simulink model "HT_ctrl_MPC_23"  (R2023a)
settings: Solver=VariableStepAuto  StartTime=0.0  StopTime=50  FixedStep=1  RelTol=1e-3
undefined symbols (not defined in the file): D1, Delta, robust_actuator_gain_scale, robust_actuator_rate_limit, robust_actuator_time_constant, robust_load_switch_time, robust_measurement_delay_s, robust_noise_seed, robust_noise_std
libraries: spsThreePhaseParallelRLCLoadLib x3, spsExcitationSystemModel x2, spsThreePhaseSourceLib x1, simulink x1, spsSynchronousMachinepuStandardLib x1, spsThreePhaseBreakerLib x1, spsThreePhaseTransformerTwoWindingsLib x1, spsVoltageMeasurementLib x1, spsGroundLib x1, spspowerguiLib x1
Description:
  | Phase-2.3 filtered, disturbance-estimating MPC with soft output constraints and anti-windup; generated from phase-2 harness.
settings Model: Creator=zzzaa  LastModifiedBy=User
settings OptimizationCC: ReuseModelBlockBuffer=off

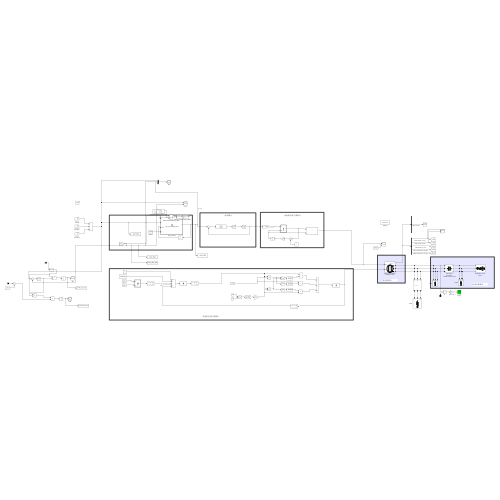
[thumbnail: Simulink's stored preview of the top-level diagram]
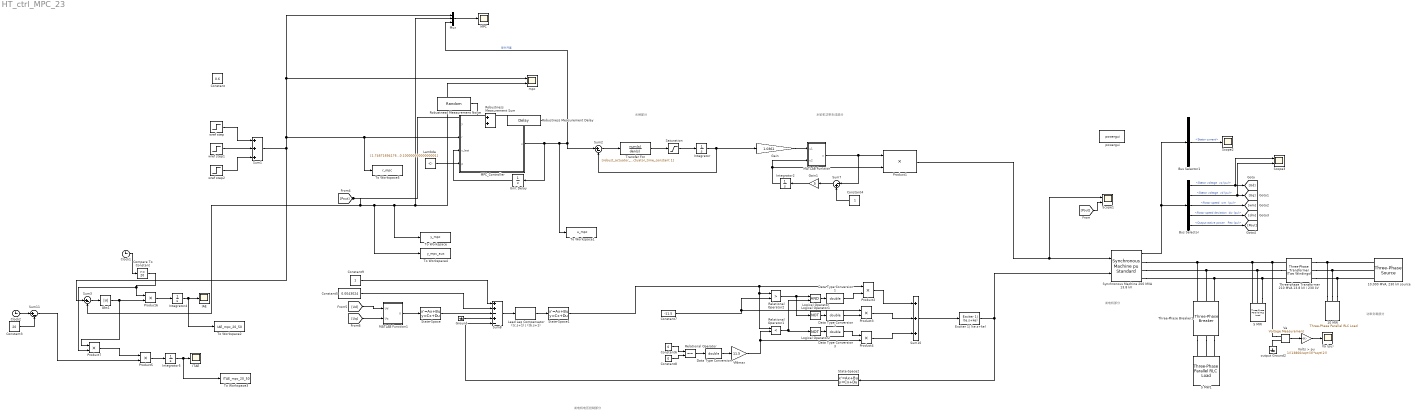
== system HT_ctrl_MPC_23 ==
  note: 水轮机功率生成部分
  note: 水闸部分
  note: 发电机电压控制部分
  note: 发电机部分
  note: 功率负载部分
  10 MW : spsThreePhaseParallelRLCLoadLib/Three-Phase Parallel RLC Load  LConnTagsString=A|B|C  Configuration=Y (grounded)  NominalVoltage=230e3  Vabc=[1e3 1e3 1e3]  Vabcp=[1e3 1e3 1e3]  NominalFrequency=60  UnbalancedPower=off  ActivePower=10000000  InductivePower=0  CapacitivePower=0  Pabc=[10e3 9e3 11e3]  QLabc=[100 90 110]  QCabc=[100 90 110]  Pabcp=[10e3 9e3 11e3]  QLabcp=[100 90 110]  QCabcp=[100 90 110]  Measurements=None  LoadType=constant Z
  "10,000 MVA, 230 kV source" : spsThreePhaseSourceLib/Three-Phase Source  InternalConnection=Yg  VoltagePhases=off  Voltage=(230000)*1.00006  PhaseAngle=-0.77547  Voltage_phases=[25e3 25e3 25e3]/sqrt(3)  PhaseAngles_phases=[0 -120 +120]  Frequency=60  NonIdealSource=on  SpecifyImpedance=on  Resistance=0.529  Inductance=0.0140  ShortCircuitLevel=10000e6  BaseVoltage=230e3  XRratio=10  BusType=swing  Pref=0  Qref=0  Prefabc=[10e3, 10e3, 10e3]  Qrefabc=[0, 0, 0]  Qmin=-Inf  Qmax=Inf
  5 MW : spsThreePhaseParallelRLCLoadLib/Three-Phase Parallel RLC Load  LConnTagsString=A|B|C  Configuration=Y (grounded)  NominalVoltage=13.8e3  Vabc=[1e3 1e3 1e3]  Vabcp=[1e3 1e3 1e3]  NominalFrequency=60  UnbalancedPower=off  ActivePower=5000000  InductivePower=0  CapacitivePower=0  Pabc=[10e3 9e3 11e3]  QLabc=[100 90 110]  QCabc=[100 90 110]  Pabcp=[10e3 9e3 11e3]  QLabcp=[100 90 110]  QCabcp=[100 90 110]  Measurements=None  LoadType=constant Z
  5 MW1 : spsThreePhaseParallelRLCLoadLib/Three-Phase Parallel RLC Load  LConnTagsString=A|B|C  Configuration=Y (grounded)  NominalVoltage=13.8e3  Vabc=[1e3 1e3 1e3]  Vabcp=[1e3 1e3 1e3]  NominalFrequency=60  UnbalancedPower=off  ActivePower=robust_load_power_w  InductivePower=0  CapacitivePower=0  Pabc=[10e3 9e3 11e3]  QLabc=[100 90 110]  QCabc=[100 90 110]  Pabcp=[10e3 9e3 11e3]  QLabcp=[100 90 110]  QCabcp=[100 90 110]  Measurements=None  LoadType=constant Z
  Abs1 : Abs  ZeroCross=off  SaturateOnIntegerOverflow=off
  Bus Selector : BusSelector  OutputSignals="dq0 components.Stator voltage  vq (pu),dq0 components.Stator voltage  vd (pu),Mechanical.Rotor speed  wm  (pu),Mechanical.Rotor speed deviation  dw (pu),Output active power   Peo (pu)"
  Bus Selector1 : BusSelector  OutputSignals=Stator current
  Clock1 : Clock
  Clock2 : Clock
  Compare To Constant : simulink/Logic and Bit Operations/Compare To Constant  relop=>=  const=20  OutDataTypeStr=boolean
  Constant : Constant  Value=0.6
  Constant3 : Constant  Value=20
  Constant4 : Constant
  Constant5 : Constant  Value=0.0043024
  Constant6 : Constant  Value=0
  Constant7 : Constant  Value=-11.5
  Constant8 : Constant  Value=0
  Constant9 : Constant
  Data Type Conversion{,1..3} (4 alike) : DataTypeConversion  OutDataTypeStr=double  SaturateOnIntegerOverflow=off  RndMeth=Floor
  Exciter 1| (te.s+ke) : spsExcitationSystemModel/Continuous/Exciter 1| (te.s+ke)  N=1  D=[0 1]  Y0=1.2907  U0=1.2907
  Gain : Gain  Gain=1.0361
  Gain1 : Gain  Gain=5
  Ground : Ground
  IAE : Scope
  ITAE : Scope
  Integrator : Integrator  InitialCondition=0.72544  LimitOutput=on  UpperSaturationLimit=0.97518  LowerSaturationLimit=0.01
  Integrator2 : Integrator  InitialCondition=0.75161
  Integrator4 : Integrator
  Integrator5 : Integrator
  Lambda : Constant  Value=[1.7467169417629138 -0.75577185457135487 0.064765752859370848 -0.055077765078686149 -0.00021442550980328465 1 40 0.014999999999999999 -1.1499999999999999 1.1499999999999999 0.029999999999999999 0.029999999999999999 0.02 0.10000000000000001 0.050000000000000003 0.02 0.34999999999999998 1 20 0.10000000000000001]
  Lead Lag Compensator (tc.s+1) | (tb.s+1) : spsExcitationSystemModel/Continuous/Lead Lag Compensator (tc.s+1) | (tb.s+1)  N=[0 1]  D=[0 1]  Y0=0.0043024  U0=0.0043024
  Logical Operator : Logic
  Logical Operator1 : Logic  Operator=NOT  Inputs=1
  Logical Operator2 : Logic  Operator=NOT  Inputs=1
  MATLAB Function : MATLAB Function  TreatAsAtomicUnit=on
  MATLAB Function1 : MATLAB Function  TreatAsAtomicUnit=on
  MPC : Scope
  MPC_Controller : MATLAB Function  TreatAsAtomicUnit=on  SystemSampleTime=0.01
  Mux : Mux  Inputs=3
  Product{1,5..7} (4 alike) : Product
  Product2 : Product  InputSameDT=on  SaturateOnIntegerOverflow=on  OutDataTypeStr=Inherit: Same as first input
  Product3 : Product  InputSameDT=on  SaturateOnIntegerOverflow=on  OutDataTypeStr=Inherit: Same as first input
  Product4 : Product  InputSameDT=on  SaturateOnIntegerOverflow=on  OutDataTypeStr=Inherit: Same as first input
  Relational Operator : RelationalOperator  Operator===
  Relational Operator1 : RelationalOperator  Operator=<
  Relational Operator2 : RelationalOperator  Operator=>
  Robustness Measurement Delay : TransportDelay  DelayTime=robust_measurement_delay_s  InitialOutput=0.5
  Robustness Measurement Noise : RandomNumber  Variance=robust_noise_std^2  Seed=robust_noise_seed  SampleTime=0.01
  Robustness Measurement Sum : Sum
  Saturation : Saturate  UpperLimit=robust_actuator_rate_limit  LowerLimit=-robust_actuator_rate_limit
  Scope1 : Scope  NumInputPorts=2
  Scope2 : Scope
  Scope3 : Scope  NumInputPorts=2
  State-Space : StateSpace  A=-50  C=50  D=0  InitialCondition=0.02
  State-Space1 : StateSpace  A=-1000  C=300000  D=0  InitialCondition=4.3024e-6
  State-Space2 : StateSpace  A=-10  C=-0.1  D=0.01  InitialCondition=0.1297
  Sum1 : Sum  Inputs=+++  InputSameDT=on  SaturateOnIntegerOverflow=on  OutDataTypeStr=Inherit: Same as first input
  Sum10 : Sum  Inputs=+++  InputSameDT=on  SaturateOnIntegerOverflow=on  OutDataTypeStr=Inherit: Same as first input
  Sum11 : Sum  Inputs=|+-
  Sum2 : Sum  Inputs=|+-
  Sum3 : Sum  Inputs=|+-
  Sum7 : Sum  Inputs=|-+
  Sum8 : Sum  Inputs=++-+-  InputSameDT=on  SaturateOnIntegerOverflow=on  OutDataTypeStr=Inherit: Same as first input
  Synchronous Machine 200 MVA 13.8 kV : spsSynchronousMachinepuStandardLib/Synchronous Machine pu Standard  PresetModel=No  MechanicalLoad=Mechanical power Pm  ShowDetailedParameters=on  RotorType=Salient-pole  Units=per unit standard parameters  MeasurementBus=off  NominalParameters="[ 200E6  13800   60 ]"  Reactances1=[ 31 32 33 34 35 36 37 ]  Reactances2=[ 1.305, 0.296, 0.252, 0.474, 0.243, 0.18 ]  dAxisTimeConstants=Short-circuit  qAxisTimeConstants=Open-circuit  TimeConstants1=[]  TimeConstants2=[]  TimeConstants3=[]  TimeConstants4=[]  TimeConstants5=[ 1.01, 0.053, 0.1 ]  TimeConstants6=[]  TimeConstants7=[]  TimeConstants8=[]  StatorResistance=2.8544e-3  Mechanical=[ 3.2 0 2]  PolePairs=2  InitialConditions=[0 -94.2826 0.750185 0.750185 0.750185 -24.943 -144.943 95.057 1.29071]  SetSaturation=off  Saturation=[0.6404,0.7127,0.8441,0.9214,0.9956,1.082,1.19,1.316,1.457;0.7,0.7698,0.8872,0.9466,0.9969,1.046,1.1,1.151,1.201]  LoadFlowParameters=[1 150000000 0 0]  TsPowergui=0  TsBlock=-1  IterativeModel=Trapezoidal non iterative  IterativeDiscreteModel=Trapezoidal non iterative  BusType=PV  Pref=150000000  Qref=0  Qmin=-Inf  Qmax=Inf  PLF=0  QLF=0
  Three-Phase Breaker1 : spsThreePhaseBreakerLib/Three-Phase Breaker  InitialState=open  SwitchA=on  SwitchB=on  SwitchC=on  SwitchTimes=[robust_load_switch_time]  External=off  BreakerResistance=0.01  SnubberResistance=1e6  SnubberCapacitance=inf  Measurements=None
  Three-phase Transformer 210 MVA 13.8 kV / 230 kV : spsThreePhaseTransformerTwoWindingsLib/Three-Phase Transformer (Two Windings)  Winding1Connection=Delta (D1)  Winding2Connection=Yg  CoreType=Three single-phase transformers  SetSaturation=off  Hysteresis=off  DataFile='hysteresis'  SetInitialFlux=off  Measurements=None  UNITS=pu  NominalPower=[ 210e6 60 ]  Winding1="[ 13.8e3 0.0027  0.08]"  Winding2=[ 230e3 0.0027 0.08]  Rm=500  Lm=500  L0=0.5  Saturation="[ 0,0  ;  0.005,1.2  ;  1.0,1.4 ]"  InitialFluxes=[ 0.8 , -0.8 , 0.7 ]  BreakLoop=off  DiscreteSolver=Trapezoidal iterative  DataType=off  TransfoNumber=0
  To Workspace : ToWorkspace  VariableName=y_mpc  SampleTime=-1
  To Workspace1 : ToWorkspace  VariableName=u_mpc  SampleTime=-1
  To Workspace2 : ToWorkspace  VariableName=IAE_mpc_20_50  SampleTime=-1
  To Workspace3 : ToWorkspace  VariableName=ITAE_mpc_20_50  SampleTime=-1
  To Workspace4 : ToWorkspace  VariableName=y_mpc_aux  SampleTime=-1
  To Workspace5 : ToWorkspace  VariableName=r_mpc  SampleTime=-1
  Transfer Fcn : TransferFcn  Numerator=[robust_actuator_gain_scale*10/3]  Denominator=[robust_actuator_time_constant 1]
  Unit Delay : UnitDelay  SampleTime=0.01  HasFrameUpgradeWarning=on
  Va : spsVoltageMeasurementLib/Voltage Measurement  Tag=PoWeRsYsTeMmEaSuReMeNt  PhasorSimulation=off  OutputType=Magnitude  PSBequivalent=0
  Va (pu) : Scope
  Vfdmax : Gain  Gain=11.5  SaturateOnIntegerOverflow=on  OutDataTypeStr=Inherit: Same as input  ParamDataTypeStr=Inherit: Same as input
  Volts > pu : Gain  Gain=1/(13800/sqrt(3)*sqrt(2))  SaturateOnIntegerOverflow=on  OutDataTypeStr=Inherit: Same as input  ParamDataTypeStr=Inherit: Same as input
  mpc : Scope  NumInputPorts=2
  output Ground2 : spsGroundLib/Ground  LConnTagsString=a
  powergui : spspowerguiLib/powergui  Priority=2  SimulationMode=Continuous  SampleTime=0  frequency=60  Iterations=50  frequencyindice=60  Pbase=100e6  ErrMax=0.0001  UnitsV=kV  UnitsW=MW  buscounter=0  FunctionMessages=off  echomessages=off  EnableUseOfTLC=off  CurrentSourceSwitches=off  DisableSnubberDevices=off  DisableRonSwitches=off  DisableVfSwitches=off  DisplayEquations=off  AutomaticDiscreteSolvers=off  SolverType=Tustin  Interpol=off  ExternalGateDelay=off  methode=off  Ts=0  x0status=blocks  SPID=on  SwTol=0  HookPort=off  NonlinearTolerance=0  nMaxIteration=15  ContinueOnMaxIteration=off  RestoreLinks=warning  ResistiveCurrentMeasurement=off  Frange=logspace(0,3,50)  Ylog=off  Xlog=off  ShowGrid=off  save=off  variable=ZData  structure=0  ZoomFFT=on  StartTime=0.0  cycles=2  DisplayStyle=off  fundamental=60  FreqAxis=off  MaxFrequency=1000  frequencyindicesteady=1  RmsSteady=1  display=off
  wref step : Step  Time=0  After=0.5  SampleTime=0
  wref step1 : Step  Time=20  After=0.25  SampleTime=0
  wref step2 : Step  Time=35  After=0.15  SampleTime=0
  wires:
  Va/1 -> Volts > pu/1
  Volts > pu/1 -> Va (pu)/1
  Synchronous Machine 200 MVA 13.8 kV/1 -> Bus Selector1/1, Bus Selector/1
  Bus Selector/1 -> Scope3/1, [Ud]  "<Stator voltage  vq (pu)>"
  Bus Selector/2 -> Scope3/2, [Uq]  "<Stator voltage  vd (pu)>"
  Bus Selector/3 -> [wm]  "<Rotor speed  wm  (pu)>"
  Bus Selector/4 -> [dm]  "<Rotor speed deviation  dw (pu)>"
  Bus Selector/5 -> [Pout]  "<Output active power   Peo (pu)>"
  MPC_Controller/1(u) -> To Workspace1/1, Sum2/1, Mux/3, Unit Delay/1  "导叶开度"
  Transfer Fcn/1 -> Saturation/1
  Saturation/1 -> Integrator/1
  Sum2/1 -> Transfer Fcn/1
  Gain/1 -> MATLAB Function/1(u1)
  MATLAB Function/1(y) -> Product1/1, Sum7/1
  Constant4/1 -> Sum7/2
  Sum7/1 -> Gain1/1
  Gain1/1 -> Integrator2/1
  Integrator2/1 -> MATLAB Function/2(u2), Product1/2
  State-Space2/1 -> Sum8/5
  Exciter 1| (te.s+ke)/1 -> Synchronous Machine 200 MVA 13.8 kV/2, State-Space2/1
  MATLAB Function1/1(U) -> State-Space/1
  Lead Lag Compensator (tc.s+1) | (tb.s+1)/1 -> State-Space1/1
  [Ud] -> MATLAB Function1/1(Ud)
  Constant5/1 -> Sum8/2
  Constant9/1 -> Sum8/1
  Sum10/1 -> Exciter 1| (te.s+ke)/1
  [Uq] -> MATLAB Function1/2(Uq)
  Sum8/1 -> Lead Lag Compensator (tc.s+1) | (tb.s+1)/1
  Ground/1 -> Sum8/4
  Logical Operator2/1 -> Data Type Conversion3/1
  State-Space/1 -> Sum8/3
  Constant6/1 -> Relational Operator/1
  Product2/1 -> Sum10/1
  Constant8/1 -> Relational Operator/2
  Product4/1 -> Sum10/3
  Relational Operator1/1 -> Logical Operator2/1, Logical Operator/2
  Product3/1 -> Sum10/2
  Constant7/1 -> Product3/1, Relational Operator2/2
  Relational Operator2/1 -> Logical Operator1/1, Logical Operator/1
  Logical Operator/1 -> Data Type Conversion1/1
  Vfdmax/1 -> Product4/2, Relational Operator1/2
  State-Space1/1 -> Product2/1, Relational Operator1/1, Relational Operator2/1
  Data Type Conversion/1 -> Vfdmax/1
  Data Type Conversion1/1 -> Product2/2
  Data Type Conversion2/1 -> Product3/2
  Logical Operator1/1 -> Data Type Conversion2/1
  Data Type Conversion3/1 -> Product4/1
  Relational Operator/1 -> Data Type Conversion/1
  Product1/1 -> Scope1/1, Synchronous Machine 200 MVA 13.8 kV/1
  Bus Selector1/1 -> Scope2/1  "<Stator current>"
  [Pout] -> Scope1/2
  wref step/1 -> Sum1/1
  wref step1/1 -> Sum1/2
  wref step2/1 -> Sum1/3
  Mux/1 -> MPC/1
  Integrator/1 -> Sum2/2, Gain/1
  Unit Delay/1 -> MPC_Controller/3(u_last)
  Clock1/1 -> Compare To Constant/1
  Compare To Constant/1 -> Product7/2, Product6/1
  Clock2/1 -> Sum11/1
  Product7/1 -> Product5/1
  Sum11/1 -> Product5/2
  Product6/1 -> Integrator4/1
  Constant3/1 -> Sum11/2
  Sum3/1 -> Abs1/1
  Integrator4/1 -> To Workspace2/1, IAE/1
  Sum1/1 -> Sum3/1, mpc/1, Mux/1, MPC_Controller/2(r), To Workspace5/1
  Product5/1 -> Integrator5/1
  Integrator5/1 -> To Workspace3/1, ITAE/1
  [Pout] -> Sum3/2, To Workspace4/1, To Workspace/1, Mux/2, mpc/2, Robustness Measurement Sum/1
  Abs1/1 -> Product7/1, Product6/2
  Lambda/1 -> MPC_Controller/4(p)
  Robustness Measurement Noise/1 -> Robustness Measurement Sum/2
  Robustness Measurement Sum/1 -> Robustness Measurement Delay/1
  Robustness Measurement Delay/1 -> MPC_Controller/1(y)
  connections:
  10 MW/LConn2 -- Three-phase Transformer 210 MVA 13.8 kV / 230 kV/RConn2 -- "10,000 MVA, 230 kV source"/RConn2
  Va/LConn1 -- Three-Phase Breaker1/LConn1 -- Synchronous Machine 200 MVA 13.8 kV/RConn1 -- 5 MW/LConn1 -- Three-phase Transformer 210 MVA 13.8 kV / 230 kV/LConn1
  10 MW/LConn3 -- Three-phase Transformer 210 MVA 13.8 kV / 230 kV/RConn3 -- "10,000 MVA, 230 kV source"/RConn3
  10 MW/LConn1 -- Three-phase Transformer 210 MVA 13.8 kV / 230 kV/RConn1 -- "10,000 MVA, 230 kV source"/RConn1
  5 MW/LConn3 -- Three-Phase Breaker1/LConn3 -- Synchronous Machine 200 MVA 13.8 kV/RConn3 -- Three-phase Transformer 210 MVA 13.8 kV / 230 kV/LConn3
  Three-phase Transformer 210 MVA 13.8 kV / 230 kV/LConn2 -- Synchronous Machine 200 MVA 13.8 kV/RConn2 -- Three-Phase Breaker1/LConn2 -- 5 MW/LConn2
  output Ground2/LConn1 -- Va/LConn2
  Three-Phase Breaker1/RConn3 -- 5 MW1/LConn3
  Three-Phase Breaker1/RConn2 -- 5 MW1/LConn2
  Three-Phase Breaker1/RConn1 -- 5 MW1/LConn1

== matlab function HT_ctrl_MPC_23/MATLAB Function1 ==
  data: Ud input; U output; Uq input
function U = fcn(Ud, Uq)

U = sqrt(Ud^2+Uq^2);

== matlab function HT_ctrl_MPC_23/MATLAB Function ==
  data: u1 input; y output; u2 input
function y = fcn(u1,u2)

y = (u2/u1)^2;

end

== matlab function HT_ctrl_MPC_23/MPC_Controller ==
  data: y input; r input; u output; u_last input; p input
function u = mpc_23_controller_block(y, r, u_last, p)
%#codegen
% Phase-2.3 fixed-model MPC. Plant: 0.01 s; optimizer: 0.05 s.
% p(1:14) are the frozen phase-1 parameters. Added settings are:
% [measurement_alpha, disturbance_alpha, output_min, output_max,
%  soft_output_weight, antiwindup_decay].

persistent y_previous held_input move_plan prediction_free prediction_moves
persistent hessian gradient_step sample_counter filtered_reference
persistent filtered_measurement integral_trim previous_reference gate_counter
persistent disturbance_estimate predicted_next_output initialized
persistent filter_fast_counter

prediction_horizon = 40;
control_horizon = 4;
iterations = 20;
execution_divider = 5;

if isempty(initialized)
    a1 = p(1); a2 = p(2); b1 = p(3); b2 = p(4); bias = p(5);
    output_weight = p(6); move_weight = p(7);
    state_matrix = [ ...
        a1, a2, b1 + b2, bias; ...
        1.0, 0.0, 0.0, 0.0; ...
        0.0, 0.0, 1.0, 0.0; ...
        0.0, 0.0, 0.0, 1.0];
    input_matrix = [b1; 0.0; 1.0; 0.0];
    output_matrix = [1.0, 0.0, 0.0, 0.0];
    prediction_free = zeros(40, 4);
    prediction_moves = zeros(40, 4);
    state_power = eye(4);
    impulse_response = zeros(40, 1);
    for prediction_step = 1:prediction_horizon
        state_power = state_power * state_matrix;
        prediction_free(prediction_step, :) = output_matrix * state_power;
        if prediction_step == 1
            impulse_response(prediction_step) = output_matrix * input_matrix;
        else
            impulse_response(prediction_step) = ...
                prediction_free(prediction_step - 1, :) * input_matrix;
        end
    end
    for prediction_step = 1:prediction_horizon
        for move_index = 1:control_horizon
            response_index = prediction_step - move_index + 1;
            if response_index >= 1
                prediction_moves(prediction_step, move_index) = ...
                    impulse_response(response_index);
            end
        end
    end
    hessian = 2.0 * (output_weight * ...
        (prediction_moves' * prediction_moves) + ...
        move_weight * eye(control_horizon));
    % Include the worst-case curvature of the squared soft-output penalty.
    gradient_step = 0.8 / max(max(sum(abs(hessian), 2)) + ...
        2.0 * p(19) * max(max(sum(abs(prediction_moves' * ...
        prediction_moves), 2)), 0), 1e-9);

    y_previous = y;
    held_input = u_last;
    move_plan = zeros(4, 1);
    sample_counter = 0;
    filtered_reference = r;
    filtered_measurement = y;
    integral_trim = 0.0;
    previous_reference = r;
    gate_counter = 0;
    disturbance_estimate = 0.0;
    predicted_next_output = y;
    filter_fast_counter = 0;
    initialized = true;
end

if sample_counter > 0
    sample_counter = sample_counter - 1;
    u = held_input;
    return;
end
sample_counter = execution_divider - 1;

output_weight = p(6);
du_limit = p(8);
u_min = p(9); u_max = p(10);
integral_gain = p(11); integral_limit = p(12);
integration_gate = p(13); reference_filter_alpha = p(14);
measurement_alpha = p(15); disturbance_alpha = p(16);
output_min = p(17); output_max = p(18);
soft_output_weight = p(19); antiwindup_decay = p(20);

if abs(r - previous_reference) > 1e-8
    integral_trim = 0.0;
    gate_counter = 0;
    filter_fast_counter = 80;
end
previous_reference = r;
% Follow set-point changes for four seconds at a fast bandwidth. At steady
% operation use the stronger low-pass setting to suppress sensor noise.
if filter_fast_counter > 0 || ...
        abs(r - filtered_measurement) > 1.5 * integration_gate
    active_measurement_alpha = 0.8;
else
    active_measurement_alpha = measurement_alpha;
end
filter_fast_counter = max(filter_fast_counter - 1, 0);
% Filter only the controller measurement; the plant output and evaluation
% signals remain unfiltered. Filter state is retained between MPC updates.
filtered_measurement = filtered_measurement + ...
    active_measurement_alpha * (y - filtered_measurement);
filtered_reference = filtered_reference + ...
    reference_filter_alpha * (r - filtered_reference);

% Innovation from the preceding one-step prediction estimates a constant
% additive output disturbance. Bound it to avoid reacting to large steps.
innovation = filtered_measurement - predicted_next_output;
disturbance_estimate = disturbance_estimate + ...
    disturbance_alpha * innovation;
disturbance_estimate = max(-integral_limit, ...
    min(disturbance_estimate, integral_limit));

tracking_error = r - filtered_measurement;
pushing_high = held_input >= u_max - du_limit && tracking_error > 0;
pushing_low = held_input <= u_min + du_limit && tracking_error < 0;
pushing_output_high = filtered_measurement >= output_max && ...
    tracking_error > 0;
pushing_output_low = filtered_measurement <= output_min && ...
    tracking_error < 0;
if pushing_high || pushing_low || pushing_output_high || pushing_output_low
    % Unwind the accumulated target correction when a limit prevents the
    % requested action. In the interior, preserve phase-1 gated integration.
    integral_trim = (1.0 - antiwindup_decay) * integral_trim;
    gate_counter = 0;
elseif abs(tracking_error) <= integration_gate
    gate_counter = min(gate_counter + 1, 11);
    if gate_counter > 10
        integral_trim = integral_trim + integral_gain * tracking_error;
        integral_trim = max(-integral_limit, ...
            min(integral_trim, integral_limit));
    end
else
    gate_counter = 0;
end

state = [filtered_measurement; y_previous; held_input; 1.0];
corrected_reference = filtered_reference + integral_trim;
reference = corrected_reference * ones(prediction_horizon, 1);
free_output = prediction_free * state + disturbance_estimate;
free_error = free_output - reference;
gradient_offset = 2.0 * output_weight * ...
    (prediction_moves' * free_error);

for iteration = 1:iterations
    predicted_output = free_output + prediction_moves * move_plan;
    soft_violation = max(predicted_output - output_max, 0.0) + ...
        min(predicted_output - output_min, 0.0);
    soft_gradient = 2.0 * soft_output_weight * ...
        (prediction_moves' * soft_violation);
    move_plan = move_plan - gradient_step * ...
        (hessian * move_plan + gradient_offset + soft_gradient);
    cumulative_input = held_input;
    for move_index = 1:control_horizon
        move_plan(move_index) = max(-du_limit, ...
            min(move_plan(move_index), du_limit));
        proposed_input = cumulative_input + move_plan(move_index);
        if proposed_input > u_max
            move_plan(move_index) = u_max - cumulative_input;
        elseif proposed_input < u_min
            move_plan(move_index) = u_min - cumulative_input;
        end
        cumulative_input = cumulative_input + move_plan(move_index);
    end
end

predicted_next_output = free_output(1) + ...
    prediction_moves(1, :) * move_plan;
held_input = max(u_min, min(held_input + move_plan(1), u_max));
u = held_input;
y_previous = filtered_measurement;
move_plan(1:end-1) = move_plan(2:end);
move_plan(end) = 0.0;
end
